simulink model "EV6_LUT_FourWheel_EV6Battery77p4kWh_PowerCorrected"  (R2024a)
settings: Solver=ode4  StartTime=0  StopTime=60  FixedStep=0.001  RelTol=1e-3
PreLoadFcn:
  | VSS_BICYCLE=Simulink.Variant('Dual=0');
  | VSS_DUAL=Simulink.Variant('Dual=1');
  | Dual=1;
  | load('DriveCycle2.mat')
PostLoadFcn:
  | if any(exist('dsrtsu_mdlpostloadfcn', 'file') ~= 0), dsrtsu_mdlpostloadfcn('Execute', bdroot); end
InitFcn:
  | , if any(exist('rtifpga_mdlclblib', 'file') ~= 0), rtifpga_mdlclblib('Init', bdroot); end,
  | , if any(exist('dsmpb_private', 'file') ~= 0), dsmpb_private('dsmpb_mdlclblib', 'Init', bdroot); end,
  | load('DriveCycle2.mat')
model workspace (MAT data in the model file):
  DiffRatio = 10.65
  EV6_2023_BattBranchCapacity_Ah = 55.5236728838
  EV6_2023_BattEnergy_kWh = 77.4
  EV6_2023_BattNominalVoltage_V = 697
  EV6_2023_BattNumCellsParallel = 2
  EV6_2023_BattNumCellsSeries = 192
  EV6_2023_BattOpenVoltCapBpts = [0 0.1 0.2 0.3 0.4 0.5 0.6 0.7 0.8 0.9 1]
  EV6_2023_BattOpenVoltTbl = [2.96762142548 3.40364281191 3.47417488548 3.54470541822 3.61523441014 3.68576186124 3.75628777151 3.82681214095 3.94527005036 4.07101207308 4.2120755254]
  EV6_2023_BattPackCapacity_Ah = 111.047345768
  EV6_2023_BattResistSocBpts = [0 0.2 0.4 0.6 0.8 1]
  EV6_2023_BattResistTbl = [0.0163620057716 0.0118174152018 0.00807187352333 0.00375663957972 0.00266904525531 0.00103635901355 0.0019014404175 0.0172368903217 0.0121226074867 0.00758541551769 0.00474065349228 0.00337561163613 ... (42 elements, 7x6)]
  EV6_2023_BattResistTempBpts = [243.1 253.1 263.1 273.1 283.1 298.1 313.1]
  EV6_2023_InitialPackOCV_V = 726.471714233
  EV6_2023_InitialSOC = 0.638878863672
  EV6_BattCellCapacity_Ah = 60.3
  EV6_BattInitialSOC = 0.638878863672
  EV6_BattOCV_Cell_V = [2.96762142548 3.40364281191 3.47417488548 3.54470541822 3.61523441014 3.68576186124 3.75628777151 3.82681214095 3.94527005036 4.07101207308 4.2120755254]
  EV6_BattOCV_SOC = [0 0.1 0.2 0.3 0.4 0.5 0.6 0.7 0.8 0.9 1]
  EV6_BattPackCapacity_Ah = 120.6
  EV6_BattParallelCells = 2
  EV6_BattResistanceSOC = [0 0.2 0.4 0.6 0.8 1]
  EV6_BattResistanceTable_Ohm = [0.0163620057716 0.0118174152018 0.00807187352333 0.00375663957972 0.00266904525531 0.00103635901355 0.0019014404175 0.0172368903217 0.0121226074867 0.00758541551769 0.00474065349228 0.00337561163613 ... (42 elements, 7x6)]
  EV6_BattResistanceTemp_K = [243.1 253.1 263.1 273.1 283.1 298.1 313.1]
  EV6_BattSeriesCells = 192
  EV6_FinalDriveRatio = 10.65
  EV6_TargetPackResistance_Ohm = 0.132763804608
  Gas = 0.383333333333
undefined symbols (not defined in the file): accel_bp_mps2, AccelCmd, ActTqLF_Nm_, ActTqLR_Nm_, ActTqRF_Nm_, ActTqRR_Nm_, BattChargeLimitMaxPwr, BattChargeLimitSocBpts, BattChargeLimitTbl, BattDischargeLimitSocBpts, BattDischargeLimitTbl, BattDischargeMaxPwr, BrakeMaxPrs, BrakeMaxTrq, ChassisDistCg2FrontAxle, ChassisDistCg2RearAxle, ChassisVehMass, CltchCmd, CoastDown, DecelCmd, DiscIntNeverNeededParam, EnvGravCnst, EnvPrs, EnvTemp, EV6_RegenTorqueGain, EV6_TractionTorqueGain, front_share_regen_3d, front_share_traction_3d, FuelSpecificGrav, GearCmd, h, InitStates, lgSw, limitedMCT, MCT, MtrEffSpdBpts, MtrEffTbl, MtrEffTrqBpts, MtrPwrMax, MtrTrqMax, out_1, pMCT, RealSimPara, Ref_speed, Ref_time, regen_torque_bp_Nm, speed_bp_kph, SteeringCmd, SupvsryCtrlRegenBrkCutOffTbl, SupvsryCtrlRegenSpdBpts, TestScnrioCycleNum, traction_torque_bp_Nm, US06, VEH
libraries: VSIGenLib x65, simulink x54, etargetslib x38, dsmpblib x24, vehdynlibtire x12, autolibshared x11, vehdynlibsuspension x7, vehdynlibtirecommon x7, autolibpowerinfoutils x6, autolibutils x5, autolibsharedcoupling x4, autolibmappedmotor x4
(part 12 of 19)

== system EV6_LUT_FourWheel_EV6Battery77p4kWh_PowerCorrected/Vehicle Under Test1/Vehicle/Driver and Drive Cycle/Driver and PI with FF Control/Speed controller set/In-house CAVE/In-house Speed Controller ==
  note: ToDo: Maybe do something clever with FF and Brake, or maybe not.
      | Bleed FF based on refspd derivative
  RefSpd : Inport
  VehicleSpeed : Inport  Port=2
  Add : Sum  Inputs=+-
  Compare To Constant1 : simulink/Logic and Bit Operations/Compare To Constant  relop=<=  const=0.1  OutDataTypeStr=boolean  ZeroCross=off
  Compare To Constant3 : simulink/Logic and Bit Operations/Compare To Constant  relop=<=  const=0  OutDataTypeStr=boolean  ZeroCross=off
  Constant : Constant  Value=0
  Constant1 : Constant  Value=0
  Detect Fall Negative : simulink/Logic and Bit Operations/Detect Fall Negative  vinit=0  OutDataTypeStr=boolean
  Detect Rise Positive : simulink/Logic and Bit Operations/Detect Rise Positive  vinit=0  OutDataTypeStr=boolean
  Feedforward : Lookup_n-D  Commented=on  NumberOfTableDimensions=1  BreakpointsForDimension1="[0 10    20    30    40    50    60    70    80    90   100   110   120   130   140   150   160]"  Table="[0\t3.5\t12.5\t16\t20\t21\t22\t24.5\t26\t29.5\t32\t33\t34\t36\t37\t38\t39]"  ExtrapMethod=Clip  InternalRulePriority=Speed  RndMeth=Simplest
  Feedforward1 : Lookup_n-D  NumberOfTableDimensions=1  BreakpointsForDimension1="[0 10    20    30    40    50    60    70    80    90   100   110   120   130   140   150   160]"  Table="[0 2.6021    4.7790    6.8575    8.1555    9.4176   10.7914   12.3245   14.1570   15.9699   17.4605   19.0355   21.3079   22.8407   25.3373   26.9453   28.6975]"  ExtrapMethod=Clip  InternalRulePriority=Speed  RndMeth=Simplest
  FeedforwardGain : Gain
  Gain : Gain  Gain=-1
  Ground1 : Ground
  Integrator1 : Integrator  Commented=on
  Ki : Gain
  Kp : Gain  Gain=10
  Limits [-50,50] : Integrator  ExternalReset=either  LimitOutput=on  UpperSaturationLimit=50  LowerSaturationLimit=-50
  Logical Operator : Logic  Operator=OR  Inputs=3  AllPortsSameDT=off  OutDataTypeStr=boolean
  Lowpass Filter : TransferFcn  Denominator=[.02 1]
  Memory : Memory
  Memory1 : Memory
  Min threshold for Brake switch : Constant  Value=0
  Product1 : Product  RndMeth=Zero
  Proportional Gain Scheduling : Lookup_n-D  NumberOfTableDimensions=1  BreakpointsForDimension1=[ 0 30 70]  IndexSearchMethod=Linear search  BeginIndexSearchUsingPreviousIndexResult=on  Table=[1 1 1]  ExtrapMethod=Clip  UseLastTableValue=on  RndMeth=Simplest
  Relational Operator : RelationalOperator  Operator=>  OutDataTypeStr=boolean  InputSameDT=off
  Scope : Scope  NumInputPorts=2
  Scope1 : Scope
  Scope2 : Scope  NumInputPorts=3
  Scope3 : Scope
  Scope4 : Scope  NumInputPorts=2
  Sum : Sum  Inputs=|+-
  Sum1 : Sum  Inputs=+++
  Switch{1..4} (4 alike) : Switch  Criteria=u2 > Threshold  SaturateOnIntegerOverflow=off  InputSameDT=off
  standstill brake [0,100] : Constant  Value=50
  AcceleratorPedalPos : Outport  VectorParamsAs1DForOutWhenUnconnected=off
  BrakePedalPos : Outport  Port=2  VectorParamsAs1DForOutWhenUnconnected=off
  BrakeSwitch : Outport  Port=3  VectorParamsAs1DForOutWhenUnconnected=off
  wires:
  FeedforwardGain/1 -> Sum1/3  "Driver_FdfwdTerm_pct"
  Feedforward1/1 -> FeedforwardGain/1
  Product1/1 -> Sum1/2  "Driver_PropTerm_pct"
  Proportional Gain Scheduling/1 -> Product1/2
  standstill brake [0,100]/1 -> Switch4/1
  Constant/1 -> Switch3/1
  Switch1/1 -> Memory1/1, Scope4/2, Scope2/1, Switch3/3  "AcceleratorPedalPos_pct"
  Compare To Constant1/1 -> Switch4/2, Switch3/2
  Memory1/1 -> Add/1
  Memory/1 -> Add/2
  Add/1 -> Detect Rise Positive/1, Detect Fall Negative/1
  Detect Fall Negative/1 -> Logical Operator/3
  Detect Rise Positive/1 -> Logical Operator/2
  Compare To Constant3/1 -> Logical Operator/1
  Logical Operator/1 -> Limits [-50,50]/2
  Gain/1 -> Switch2/2, Switch2/1
  Ground1/1 -> Switch1/3, Switch2/3
  Sum1/1 -> Switch1/2, Switch1/1, Scope4/1, Gain/1  "Driver_TotCmdPreLim_pct"
  Relational Operator/1 -> Scope2/3, BrakeSwitch/1  "BrakeSwitch"
  Lowpass Filter/1 -> Sum/2, Scope/1  "VS_Flt"
  Switch2/1 -> Memory/1, Scope2/2, Switch4/3, Relational Operator/1  "BrakePedalPosPre_pct"
  VehicleSpeed/1 -> Lowpass Filter/1, Scope/2, Proportional Gain Scheduling/1
  Ki/1 -> Limits [-50,50]/1, Scope3/1  "Driver_IntTerm_pct"
  Sum/1 -> Scope1/1, Ki/1, Kp/1  "SpdErr"
  RefSpd/1 -> Sum/1, Compare To Constant3/1, Compare To Constant1/1, Feedforward1/1  "RefSpd"
  Min threshold for Brake switch/1 -> Relational Operator/2
  Kp/1 -> Product1/1
  Switch3/1 -> AcceleratorPedalPos/1  "AcceleratorPedalPos_pct"
  Switch4/1 -> BrakePedalPos/1  "BrakePedalPos_pct"
  Limits [-50,50]/1 -> Sum1/1  "Driver_IntTerm_pct"

== system EV6_LUT_FourWheel_EV6Battery77p4kWh_PowerCorrected/Vehicle Under Test1/Vehicle/Driver and Drive Cycle/Driver and PI with FF Control/Speed controller set/Predictive/Longitudinal Driver1 ==
  note: To switch variants, right-click on this subsystem (from one level above) and chose:
      | Variant, Active choice, <your selection>
  "Vref " : Inport
  "Vfdbk " : Inport  Port=2
  Longitudinal Driver : Subsystem  VariantControl=0
      mask Display: image('LongitudinalDriver.png', 'center')
  Open Loop : Subsystem  VariantControl=1
      mask Display: disp('Open Loop')
  " OpCmds" : Outport  VectorParamsAs1DForOutWhenUnconnected=off

== system EV6_LUT_FourWheel_EV6Battery77p4kWh_PowerCorrected/Vehicle Under Test1/Vehicle/Driver and Drive Cycle/Driver and PI with FF Control/Speed controller set/Speed tracking controller/In-house CAVE ==
  note: BrakeSwitch
  RefSpd [km/hr] : Inport
  In2 : Inport  Port=2
  Vehicle Speed Controller : Subsystem
  AccelPedalCmd : Outport
  BrakePedalCmd : Outport  Port=2
  Out3 : Outport  Port=3
  wires:
  Vehicle Speed Controller/1(AcceleratorPedalPos) -> AccelPedalCmd/1  "AccelPedalCmd"
  In2/1 -> Vehicle Speed Controller/2(VehicleSpeed)
  RefSpd [km/hr]/1 -> Vehicle Speed Controller/1(RefSpd)
  Vehicle Speed Controller/2(BrakePedalPos) -> BrakePedalCmd/1  "BrakePedalCmd"
  Vehicle Speed Controller/3(BrakeSwitch) -> Out3/1

== system EV6_LUT_FourWheel_EV6Battery77p4kWh_PowerCorrected/Vehicle Under Test1/Vehicle/Driver and Drive Cycle/Driver and PI with FF Control/Speed controller set/Speed tracking controller/PIF ==
  RefSpd [km/hr] : Inport
  In2 : Inport  Port=2
  Compare To Constant1 : simulink/Logic and Bit Operations/Compare To Constant  relop=<=  const=0.1  OutDataTypeStr=boolean  ZeroCross=off
  Constant : Constant  Value=0
  Constant1 : Constant  Value=0
  Gain : Gain  Gain=1/3.6
  Gain1 : Gain  Gain=1/3.6
  Gain2 : Gain  Gain=100
  Gain3 : Gain  Gain=100
  Longitudinal Driver : autolibshared/Longitudinal Driver  extAccelOvr=off  extDecelOvr=off  extAccelHld=off  extDecelHld=off  extAccelZero=off  extDecelZero=off  cntrlType=PI  shftType=None  velUnits=m/s  gearOut=off  Kp=2  Ki=2  Kff=.1*0.4  Kg=0  VehVelVec=[0 100]  KffVec=[.1 .1]  KpVec=[10 10]  KiVec=[5 5]  KgVec=[0 0]  m=1500  Kpt=3000  tau=.1  L=2  aR=200  bR=2.5  cR=.5  g=9.81  vnom=1  Kaw=1  tauerr=.01  tauPt=2  GearInit=0  tShift=.1  pdlVec=[0.1 0.4 0.5 0.9]  upShftTbl=[-1 12.9375 26.4375 39.9375 51.18749999999999 62.4375 72.84375 83.25;-1 16.3125 29.8125 43.3125 54.5624 65.8125 76.78125 87.75;-1 19.6875 33.1875 46.68749999999999 57.9375 69.1875 80.71875 92.25;-1 33 52.5 77.25 100.5 138.75 161.875 185]  dwnShftTbl=[1 9.5625 23.0625 36.5625 47.8125 59.0625 68.90625 78.75;1 12.9375 26.4375 39.9375 51.18749999999999 62.4375 72.84375 83.25;1 16.3125 29.8125 43.3125 54.562499 65.8125 76.78125 87.75;1 19.6875 33.1875 46.68749999999999 57.9375 69.1875 80.71875 92.25]  tClutch=.5  tRev=.5  tPark=120  aMode=2  UpGearVec="[0  1  2  3  4  5  6  7]"  DownGearVec="[1  2  3  4  5  6  7  8]"
      settings: LibrarySourceBlock=vehdynlibdriver/Longitudinal Driver
  Lowpass Filter : TransferFcn  Denominator=[.01 1]
  Min threshold for Brake switch : Constant  Value=0
  Relational Operator : RelationalOperator  Operator=>  OutDataTypeStr=boolean  InputSameDT=off
  Switch3 : Switch  Criteria=u2 > Threshold  SaturateOnIntegerOverflow=off  InputSameDT=off
  Switch4 : Switch  Criteria=u2 > Threshold  SaturateOnIntegerOverflow=off  InputSameDT=off
  Terminator : Terminator
  standstill brake [0,1] : Constant  Value=0.5
  AccelPedalCmd : Outport
  BrakePedalCmd : Outport  Port=2
  Out3 : Outport  Port=3
  wires:
  Lowpass Filter/1 -> Gain1/1  "VS_Flt"
  Switch4/1 -> Gain3/1  "BrakePedalPos_pct"
  Switch3/1 -> Gain2/1  "AcceleratorPedalPos_pct"
  standstill brake [0,1]/1 -> Switch4/1
  Compare To Constant1/1 -> Switch3/2, Switch4/2
  Constant/1 -> Switch3/1
  Longitudinal Driver/2 -> Switch3/3  "AcceleratorPedalPosPre_pct"
  Longitudinal Driver/1 -> Terminator/1
  Gain2/1 -> AccelPedalCmd/1  "AccelPedalCmd"
  Gain3/1 -> BrakePedalCmd/1  "BrakePedalCmd"
  In2/1 -> Lowpass Filter/1
  RefSpd [km/hr]/1 -> Gain/1
  Constant1/1 -> Longitudinal Driver/3
  Gain/1 -> Longitudinal Driver/1, Compare To Constant1/1
  Longitudinal Driver/3 -> Relational Operator/1, Switch4/3  "BrakePedalPosPre_pct"
  Relational Operator/1 -> Out3/1  "BrakeSwitch"
  Min threshold for Brake switch/1 -> Relational Operator/2
  Gain1/1 -> Longitudinal Driver/2

== system EV6_LUT_FourWheel_EV6Battery77p4kWh_PowerCorrected/Vehicle Under Test1/Vehicle/Driver and Drive Cycle/Driver and PI with FF Control/Speed controller set/Speed tracking controller/Predictive ==
  RefSpd [km/hr] : Inport
  In2 : Inport  Port=2
  Compare To Constant1 : simulink/Logic and Bit Operations/Compare To Constant  relop=<=  const=0.1  OutDataTypeStr=boolean  ZeroCross=off
  Constant : Constant  Value=0
  Constant1 : Constant  Value=0
  Gain : Gain  Gain=1/3.6
  Gain1 : Gain  Gain=1/3.6
  Gain4 : Gain  Gain=100
  Gain5 : Gain  Gain=100
  Longitudinal Driver : autolibshared/Longitudinal Driver  extAccelOvr=off  extDecelOvr=off  extAccelHld=off  extDecelHld=off  extAccelZero=off  extDecelZero=off  cntrlType=Predictive  shftType=None  velUnits=m/s  gearOut=off  Kp=10  Ki=5  Kff=.1  Kg=0  VehVelVec=[0 100]  KffVec=[.1 .1]  KpVec=[10 10]  KiVec=[5 5]  KgVec=[0 0]  m=2040  Kpt=6200  tau=0.1  L=3  aR=200/10  bR=2.5/10  cR=.3  g=9.807  vnom=5  Kaw=1  tauerr=.01  tauPt=2  GearInit=0  tShift=.1  pdlVec=[0.1 0.4 0.5 0.9]  upShftTbl=[-1 12.9375 26.4375 39.9375 51.18749999999999 62.4375 72.84375 83.25;-1 16.3125 29.8125 43.3125 54.5624 65.8125 76.78125 87.75;-1 19.6875 33.1875 46.68749999999999 57.9375 69.1875 80.71875 92.25;-1 33 52.5 77.25 100.5 138.75 161.875 185]  dwnShftTbl=[1 9.5625 23.0625 36.5625 47.8125 59.0625 68.90625 78.75;1 12.9375 26.4375 39.9375 51.18749999999999 62.4375 72.84375 83.25;1 16.3125 29.8125 43.3125 54.562499 65.8125 76.78125 87.75;1 19.6875 33.1875 46.68749999999999 57.9375 69.1875 80.71875 92.25]  tClutch=.5  tRev=.5  tPark=120  aMode=2  UpGearVec="[0  1  2  3  4  5  6  7]"  DownGearVec="[1  2  3  4  5  6  7  8]"
      settings: LibrarySourceBlock=vehdynlibdriver/Longitudinal Driver
  Lowpass Filter : TransferFcn  Denominator=[.02 1]
  Min threshold for Brake switch : Constant  Value=0
  Relational Operator : RelationalOperator  Operator=>  OutDataTypeStr=boolean  InputSameDT=off
  Switch3 : Switch  Criteria=u2 > Threshold  SaturateOnIntegerOverflow=off  InputSameDT=off
  Switch4 : Switch  Criteria=u2 > Threshold  SaturateOnIntegerOverflow=off  InputSameDT=off
  Terminator : Terminator
  standstill brake [0,1] : Constant  Value=0.5
  AccelPedalCmd : Outport
  BrakePedalCmd : Outport  Port=2
  Out3 : Outport  Port=3
  wires:
  Lowpass Filter/1 -> Gain1/1  "VS_Flt"
  Longitudinal Driver/2 -> Switch3/3  "AcceleratorPedalPosPre_pct"
  Gain5/1 -> BrakePedalCmd/1  "BrakePedalCmd"
  Gain/1 -> Longitudinal Driver/1, Compare To Constant1/1
  Gain4/1 -> AccelPedalCmd/1  "AccelPedalCmd"
  Constant/1 -> Switch3/1
  Compare To Constant1/1 -> Switch3/2, Switch4/2
  Switch3/1 -> Gain4/1  "AcceleratorPedalPos_pct"
  Switch4/1 -> Gain5/1  "BrakePedalPos_pct"
  Longitudinal Driver/3 -> Relational Operator/1, Switch4/3  "BrakePedalPosPre_pct"
  standstill brake [0,1]/1 -> Switch4/1
  Longitudinal Driver/1 -> Terminator/1
  In2/1 -> Lowpass Filter/1
  RefSpd [km/hr]/1 -> Gain/1
  Constant1/1 -> Longitudinal Driver/3
  Relational Operator/1 -> Out3/1  "BrakeSwitch"
  Min threshold for Brake switch/1 -> Relational Operator/2
  Gain1/1 -> Longitudinal Driver/2

== system EV6_LUT_FourWheel_EV6Battery77p4kWh_PowerCorrected/Vehicle Under Test1/Vehicle/Powertrain Supervisory Controller /Engine Torque Command/Motor Torque Arbitration and Power Management/Power Management/Check Within Limits ==
  up : Inport
  u : Inport  Port=2
  lo : Inport  Port=3
  Compare To Zero : simulink/Logic and Bit Operations/Compare To Zero  relop=>=  OutDataTypeStr=boolean
  Compare To Zero1 : simulink/Logic and Bit Operations/Compare To Zero  relop=<=  OutDataTypeStr=boolean
  Logical Operator : Logic  AllPortsSameDT=off  OutDataTypeStr=boolean
  Saturation Dynamic1 : simulink/Discontinuities/Saturation Dynamic  OutMin=[]  OutMax=[]  OutDataTypeStr=Inherit: Same as second input  OutDataType=fixdt(1, 16)  OutScaling=2^-10  DoSatur=off
  Subtract : Sum  Inputs=+-
  Subtract1 : Sum  Inputs=-+
  InLimit : Outport  VectorParamsAs1DForOutWhenUnconnected=off
  y : Outport  Port=2  VectorParamsAs1DForOutWhenUnconnected=off
  wires:
  Saturation Dynamic1/1 -> y/1
  lo/1 -> Subtract1/2, Saturation Dynamic1/3
  up/1 -> Subtract/1, Saturation Dynamic1/1
  u/1 -> Subtract1/1, Subtract/2, Saturation Dynamic1/2
  Subtract/1 -> Compare To Zero/1
  Subtract1/1 -> Compare To Zero1/1
  Compare To Zero/1 -> Logical Operator/1
  Compare To Zero1/1 -> Logical Operator/2
  Logical Operator/1 -> InLimit/1

== system EV6_LUT_FourWheel_EV6Battery77p4kWh_PowerCorrected/Vehicle Under Test1/Vehicle/Powertrain Supervisory Controller /Engine Torque Command/Motor Torque Arbitration and Power Management/Power Management/Mech to Elec Power Estimate ==
  note: Check if Motoring
      | or Generating
  note: Using an Efficiency Map, we can estimate the
      | Electric Power from the Mechanical  Torque Request.
  note: Pelec_req = Pmech_req*Eff^k,
      | k = -1 if Motoring >= 0,
      | k = 1 if Generating < 0
  MotTrqCmd : Inport
  MotSpd : Inport  Port=2
  Abs : Abs  SaturateOnIntegerOverflow=off
  Abs1 : Abs  SaturateOnIntegerOverflow=off
  Constant1 : Constant  Value=-1  SampleTime=-1
  Constant2 : Constant  SampleTime=-1
  Eff Map : Lookup_n-D  BreakpointsForDimension1=MtrEffSpdBpts  BreakpointsForDimension2=MtrEffTrqBpts  Table=MtrEffTbl  ExtrapMethod=Clip  UseLastTableValue=on  InternalRulePriority=Speed  OutDataTypeStr=Inherit: Inherit from 'Table data'  RndMeth=Simplest
      settings: InputPortMap=u0,u1
  Gain1 : Gain  Gain=1/100
  Math Function : Math  Operator=pow  SignedPower=on  OutputSignalType=real
  Product : Product
  Product3 : Product
  Product4 : Product
  Switch2 : Switch  SaturateOnIntegerOverflow=off  InputSameDT=off
  rads_to_rpm : Gain  Gain=30/pi
  MotPwrElecReq : Outport  VectorParamsAs1DForOutWhenUnconnected=off
  Eff2k : Outport  Port=2  VectorParamsAs1DForOutWhenUnconnected=off
  wires:
  Product3/1 -> Product4/1
  Switch2/1 -> Math Function/2
  Constant1/1 -> Switch2/1
  Constant2/1 -> Switch2/3
  Eff Map/1 -> Gain1/1
  Abs/1 -> Eff Map/1
  Gain1/1 -> Math Function/1
  Math Function/1 -> Eff2k/1, Product4/2
  Product4/1 -> MotPwrElecReq/1
  Abs1/1 -> Eff Map/2
  rads_to_rpm/1 -> Abs/1
  Product/1 -> Switch2/2
  MotSpd/1 -> Product3/1, Product/1, rads_to_rpm/1
  MotTrqCmd/1 -> Product3/2, Product/2, Abs1/1

== system EV6_LUT_FourWheel_EV6Battery77p4kWh_PowerCorrected/Vehicle Under Test1/Vehicle/Powertrain Supervisory Controller /Engine Torque Command/Motor Torque Arbitration and Power Management/Power Management/Torque Limit ==
  MotTrq : Inport
  MotSpd : Inport  Port=2
  Gain : Gain  Gain=-1
  Max Motor Torque : LibPtSupervisoryCtrl/Powertrain Supervisory Controller /Engine Torque Command/Accel Pedal to Traction Wheel Torque Request/Max Motor Torque  SystemSampleTime=-1  VariantActivationTime=update diagram  AllowFlexibleInterface=on  Latency=0  AutoFrameSizeCalculation=off
  Saturation Dynamic : simulink/Discontinuities/Saturation Dynamic  OutMin=[]  OutMax=[]  OutDataTypeStr=Inherit: Same as second input  OutDataType=fixdt(1, 16)  OutScaling=2^-10  DoSatur=off
  MotTrqCmd : Outport  VectorParamsAs1DForOutWhenUnconnected=off
  wires:
  MotTrq/1 -> Saturation Dynamic/2
  Saturation Dynamic/1 -> MotTrqCmd/1
  Max Motor Torque/1 -> Gain/1, Saturation Dynamic/1
  Gain/1 -> Saturation Dynamic/3
  MotSpd/1 -> Max Motor Torque/1

== system EV6_LUT_FourWheel_EV6Battery77p4kWh_PowerCorrected/Vehicle Under Test1/Vehicle/Rototest and ORNL Interface/Get Wheel Spd Cmd Based on Wheel Dynamics/Whl Dynamics & Format CM Powertrain Signal/Subsystem/WheelInertia ==
  In1 : Inport
  Divide : Product  Inputs=*/
  Switch : Switch  Criteria=u2 ~= 0  ZeroCross=off  SaturateOnIntegerOverflow=off  InputSameDT=off
  Zero : Constant
  Zero1 : Constant  Value=0.74063
  Out1 : Outport
  wires:
  Divide/1 -> Out1/1
  In1/1 -> Divide/1
  Zero/1 -> Switch/3
  Switch/1 -> Divide/2
  Zero1/1 -> Switch/2, Switch/1

== system EV6_LUT_FourWheel_EV6Battery77p4kWh_PowerCorrected/Vehicle Under Test1/Vehicle/Rototest and ORNL Interface/Get Wheel Spd Cmd Based on Wheel Dynamics/Whl Dynamics & Format CM Powertrain Signal/Subsystem/WheelInertia1 ==
  In1 : Inport
  Divide : Product  Inputs=*/
  Switch : Switch  Criteria=u2 ~= 0  ZeroCross=off  SaturateOnIntegerOverflow=off  InputSameDT=off
  Zero : Constant
  Zero1 : Constant  Value=0.82
  axleTorq : Outport
  wires:
  Divide/1 -> axleTorq/1
  In1/1 -> Divide/1
  Zero/1 -> Switch/3
  Switch/1 -> Divide/2
  Zero1/1 -> Switch/2, Switch/1

== system EV6_LUT_FourWheel_EV6Battery77p4kWh_PowerCorrected/Vehicle Under Test1/Vehicle/Rototest and ORNL Interface/Get Wheel Spd Cmd Based on Wheel Dynamics/Whl Dynamics & Format CM Powertrain Signal/Subsystem1/WheelInertia ==
  In1 : Inport
  Divide : Product  Inputs=*/
  Read CM Parameter : CarMaker4SL/Read CM Parameter  xfile=Vehicle  xkey=Wheel.fl.I  xnout=3  xdefaults=[]  xmuxed=off  xstime=Continuous
      settings: SourceProductName=CarMaker4SL
  Switch : Switch  Criteria=u2 ~= 0  ZeroCross=off  SaturateOnIntegerOverflow=off  InputSameDT=off
  Terminator : Terminator
  Terminator1 : Terminator
  Zero : Constant
  Out1 : Outport
  wires:
  Divide/1 -> Out1/1
  Read CM Parameter/1 -> Terminator/1
  Read CM Parameter/3 -> Terminator1/1
  In1/1 -> Divide/1
  Zero/1 -> Switch/3
  Switch/1 -> Divide/2
  Read CM Parameter/2 -> Switch/2, Switch/1

== system EV6_LUT_FourWheel_EV6Battery77p4kWh_PowerCorrected/Vehicle Under Test1/Vehicle/Rototest and ORNL Interface/Get Wheel Spd Cmd Based on Wheel Dynamics/Whl Dynamics & Format CM Powertrain Signal/Subsystem2/WheelInertia ==
  In1 : Inport
  Divide : Product  Inputs=*/
  Switch : Switch  Criteria=u2 ~= 0  ZeroCross=off  SaturateOnIntegerOverflow=off  InputSameDT=off
  Zero : Constant
  Zero1 : Constant  Value=0.74063
  Out1 : Outport
  wires:
  Divide/1 -> Out1/1
  In1/1 -> Divide/1
  Zero/1 -> Switch/3
  Switch/1 -> Divide/2
  Zero1/1 -> Switch/2, Switch/1

== system EV6_LUT_FourWheel_EV6Battery77p4kWh_PowerCorrected/Vehicle Under Test1/Vehicle/Rototest and ORNL Interface/Get Wheel Spd Cmd Based on Wheel Dynamics/Whl Dynamics & Format CM Powertrain Signal/Subsystem2/WheelInertia1 ==
  In1 : Inport
  Divide : Product  Inputs=*/
  Switch : Switch  Criteria=u2 ~= 0  ZeroCross=off  SaturateOnIntegerOverflow=off  InputSameDT=off
  Zero : Constant
  Zero1 : Constant  Value=0.82
  Out1 : Outport
  wires:
  Divide/1 -> Out1/1
  In1/1 -> Divide/1
  Zero/1 -> Switch/3
  Switch/1 -> Divide/2
  Zero1/1 -> Switch/2, Switch/1

== system EV6_LUT_FourWheel_EV6Battery77p4kWh_PowerCorrected/Vehicle Under Test1/Vehicle/Rototest and ORNL Interface/Get Wheel Spd Cmd Based on Wheel Dynamics/Whl Dynamics & Format CM Powertrain Signal/Subsystem3/WheelInertia ==
  In1 : Inport
  Divide : Product  Inputs=*/
  Switch : Switch  Criteria=u2 ~= 0  ZeroCross=off  SaturateOnIntegerOverflow=off  InputSameDT=off
  Zero : Constant
  Zero1 : Constant  Value=0.74063
  Out1 : Outport
  wires:
  Divide/1 -> Out1/1
  In1/1 -> Divide/1
  Zero/1 -> Switch/3
  Switch/1 -> Divide/2
  Zero1/1 -> Switch/2, Switch/1

== system EV6_LUT_FourWheel_EV6Battery77p4kWh_PowerCorrected/Vehicle Under Test1/Vehicle/Rototest and ORNL Interface/Get Wheel Spd Cmd Based on Wheel Dynamics/Whl Dynamics & Format CM Powertrain Signal/Subsystem3/WheelInertia1 ==
  In1 : Inport
  Divide : Product  Inputs=*/
  Switch : Switch  Criteria=u2 ~= 0  ZeroCross=off  SaturateOnIntegerOverflow=off  InputSameDT=off
  Zero : Constant
  Zero1 : Constant  Value=0.82
  axleTorq : Outport
  wires:
  Divide/1 -> axleTorq/1
  In1/1 -> Divide/1
  Zero/1 -> Switch/3
  Switch/1 -> Divide/2
  Zero1/1 -> Switch/2, Switch/1

== system EV6_LUT_FourWheel_EV6Battery77p4kWh_PowerCorrected/Vehicle Under Test1/Vehicle/Rototest and ORNL Interface/Get Wheel Spd Cmd Based on Wheel Dynamics/Whl Dynamics & Format CM Powertrain Signal/Subsystem4/WheelInertia ==
  In1 : Inport
  Divide : Product  Inputs=*/
  Switch : Switch  Criteria=u2 ~= 0  ZeroCross=off  SaturateOnIntegerOverflow=off  InputSameDT=off
  Zero : Constant
  Zero1 : Constant  Value=0.74063
  Out1 : Outport
  wires:
  Divide/1 -> Out1/1
  In1/1 -> Divide/1
  Zero/1 -> Switch/3
  Switch/1 -> Divide/2
  Zero1/1 -> Switch/2, Switch/1

== system EV6_LUT_FourWheel_EV6Battery77p4kWh_PowerCorrected/Vehicle Under Test1/Vehicle/Rototest and ORNL Interface/Get Wheel Spd Cmd Based on Wheel Dynamics/Whl Dynamics & Format CM Powertrain Signal/Subsystem4/WheelInertia1 ==
  In1 : Inport
  Divide : Product  Inputs=*/
  Switch : Switch  Criteria=u2 ~= 0  ZeroCross=off  SaturateOnIntegerOverflow=off  InputSameDT=off
  Zero : Constant
  Zero1 : Constant  Value=0.82
  axleTorq : Outport
  wires:
  Divide/1 -> axleTorq/1
  In1/1 -> Divide/1
  Zero/1 -> Switch/3
  Switch/1 -> Divide/2
  Zero1/1 -> Switch/2, Switch/1

== system EV6_LUT_FourWheel_EV6Battery77p4kWh_PowerCorrected/Vehicle Under Test1/Vehicle/Rototest and ORNL Interface/Get Wheel Spd Cmd Based on Wheel Dynamics/Whl Dynamics & Format CM Powertrain Signal/Subsystem5/WheelInertia1 ==
  In1 : Inport
  Divide : Product  Inputs=*/
  Read CM Parameter : CarMaker4SL/Read CM Parameter  xfile=Vehicle  xkey=Wheel.fr.I  xnout=3  xdefaults=[]  xmuxed=off  xstime=Continuous
      settings: SourceProductName=CarMaker4SL
  Switch : Switch  Criteria=u2 ~= 0  ZeroCross=off  SaturateOnIntegerOverflow=off  InputSameDT=off
  Terminator : Terminator
  Terminator1 : Terminator
  Zero : Constant
  Out1 : Outport
  wires:
  Switch/1 -> Divide/2
  Zero/1 -> Switch/3
  Read CM Parameter/2 -> Switch/1, Switch/2
  In1/1 -> Divide/1
  Read CM Parameter/3 -> Terminator1/1
  Read CM Parameter/1 -> Terminator/1
  Divide/1 -> Out1/1

== system EV6_LUT_FourWheel_EV6Battery77p4kWh_PowerCorrected/Vehicle Under Test1/Vehicle/Rototest and ORNL Interface/Get Wheel Spd Cmd Based on Wheel Dynamics/Whl Dynamics & Format CM Powertrain Signal/Subsystem6/WheelInertia2 ==
  In1 : Inport
  Divide : Product  Inputs=*/
  Read CM Parameter : CarMaker4SL/Read CM Parameter  xfile=Vehicle  xkey=Wheel.rl.I  xnout=3  xdefaults=[]  xmuxed=off  xstime=Continuous
      settings: SourceProductName=CarMaker4SL
  Switch : Switch  Criteria=u2 ~= 0  ZeroCross=off  SaturateOnIntegerOverflow=off  InputSameDT=off
  Terminator : Terminator
  Terminator1 : Terminator
  Zero : Constant
  Out1 : Outport
  wires:
  Divide/1 -> Out1/1
  Read CM Parameter/1 -> Terminator/1
  Read CM Parameter/3 -> Terminator1/1
  In1/1 -> Divide/1
  Read CM Parameter/2 -> Switch/2, Switch/1
  Zero/1 -> Switch/3
  Switch/1 -> Divide/2

== system EV6_LUT_FourWheel_EV6Battery77p4kWh_PowerCorrected/Vehicle Under Test1/Vehicle/Rototest and ORNL Interface/Get Wheel Spd Cmd Based on Wheel Dynamics/Whl Dynamics & Format CM Powertrain Signal/Subsystem7/WheelInertia3 ==
  In1 : Inport
  Divide : Product  Inputs=*/
  Read CM Parameter : CarMaker4SL/Read CM Parameter  xfile=Vehicle  xkey=Wheel.rr.I  xnout=3  xdefaults=[]  xmuxed=off  xstime=Continuous
      settings: SourceProductName=CarMaker4SL
  Switch : Switch  Criteria=u2 ~= 0  ZeroCross=off  SaturateOnIntegerOverflow=off  InputSameDT=off
  Terminator : Terminator
  Terminator1 : Terminator
  Zero : Constant
  Out1 : Outport
  wires:
  Switch/1 -> Divide/2
  Zero/1 -> Switch/3
  Read CM Parameter/2 -> Switch/1, Switch/2
  In1/1 -> Divide/1
  Read CM Parameter/3 -> Terminator1/1
  Read CM Parameter/1 -> Terminator/1
  Divide/1 -> Out1/1

== system EV6_LUT_FourWheel_EV6Battery77p4kWh_PowerCorrected/Vehicle Under Test1/Vehicle/Rototest and ORNL Interface/To Rototest with Band-Aid/Logging/RotoTestEthRXLogging/Depacker ==
  SysStsBits : Inport
  Extract Bits1 : simulink/Logic and Bit Operations/Extract Bits  bitsToExtract=Range of bits  numBits=8  bitIdxRange=[7]  outScalingMode=Preserve fixed-point scaling
  Extract Bits10 : simulink/Logic and Bit Operations/Extract Bits  bitsToExtract=Range of bits  numBits=8  bitIdxRange=[9]  outScalingMode=Preserve fixed-point scaling
  Extract Bits11 : simulink/Logic and Bit Operations/Extract Bits  bitsToExtract=Range of bits  numBits=8  bitIdxRange=[10]  outScalingMode=Preserve fixed-point scaling
  Extract Bits12 : simulink/Logic and Bit Operations/Extract Bits  bitsToExtract=Range of bits  numBits=8  bitIdxRange=[11]  outScalingMode=Preserve fixed-point scaling
  Extract Bits13 : simulink/Logic and Bit Operations/Extract Bits  bitsToExtract=Range of bits  numBits=8  bitIdxRange=[12]  outScalingMode=Preserve fixed-point scaling
  Extract Bits14 : simulink/Logic and Bit Operations/Extract Bits  bitsToExtract=Range of bits  numBits=8  bitIdxRange=[13]  outScalingMode=Preserve fixed-point scaling
  Extract Bits15 : simulink/Logic and Bit Operations/Extract Bits  bitsToExtract=Range of bits  numBits=8  bitIdxRange=[14]  outScalingMode=Preserve fixed-point scaling
  Extract Bits16 : simulink/Logic and Bit Operations/Extract Bits  bitsToExtract=Range of bits  numBits=8  bitIdxRange=[15]  outScalingMode=Preserve fixed-point scaling
  Extract Bits2 : simulink/Logic and Bit Operations/Extract Bits  bitsToExtract=Range of bits  numBits=8  bitIdxRange=[6]  outScalingMode=Preserve fixed-point scaling
  Extract Bits3 : simulink/Logic and Bit Operations/Extract Bits  bitsToExtract=Range of bits  numBits=8  bitIdxRange=[5]  outScalingMode=Preserve fixed-point scaling
  Extract Bits4 : simulink/Logic and Bit Operations/Extract Bits  bitsToExtract=Range of bits  numBits=8  bitIdxRange=[4]  outScalingMode=Preserve fixed-point scaling
  Extract Bits5 : simulink/Logic and Bit Operations/Extract Bits  bitsToExtract=Range of bits  numBits=8  bitIdxRange=[3]  outScalingMode=Preserve fixed-point scaling
  Extract Bits6 : simulink/Logic and Bit Operations/Extract Bits  bitsToExtract=Range of bits  numBits=8  bitIdxRange=[2]  outScalingMode=Preserve fixed-point scaling
  Extract Bits7 : simulink/Logic and Bit Operations/Extract Bits  bitsToExtract=Range of bits  numBits=8  bitIdxRange=[1]  outScalingMode=Preserve fixed-point scaling
  Extract Bits8 : simulink/Logic and Bit Operations/Extract Bits  bitsToExtract=Range of bits  numBits=8  bitIdxRange=[0]  outScalingMode=Preserve fixed-point scaling
  Extract Bits9 : simulink/Logic and Bit Operations/Extract Bits  bitsToExtract=Range of bits  numBits=8  bitIdxRange=[8]  outScalingMode=Preserve fixed-point scaling
  Gain : Gain  Gain=1/128
  Gain1 : Gain  Gain=1/64
  Gain10 : Gain  Gain=1/1024
  Gain11 : Gain  Gain=1/2048
  Gain12 : Gain  Gain=1/4096
  Gain13 : Gain  Gain=1/8192
  Gain14 : Gain  Gain=1/16384
  Gain15 : Gain  Gain=1/32768
  Gain2 : Gain  Gain=1/32
  Gain3 : Gain  Gain=1/16
  Gain4 : Gain  Gain=1/8
  Gain5 : Gain  Gain=1/4
  Gain6 : Gain  Gain=1/2
  Gain7 : Gain  Gain=1/1
  Gain8 : Gain  Gain=1/256
  Gain9 : Gain  Gain=1/512
  Header : VSIGenLib/Header  not=''
  Terminator{,1..11} (12 alike) : Terminator
  FaultActive : Outport
  WarningsActive : Outport  Port=2
  MeasuringStatus : Outport  Port=3
  SystemActive : Outport  Port=4
  wires:
  Extract Bits10/1 -> Gain9/1
  Extract Bits11/1 -> Gain10/1
  Extract Bits12/1 -> Gain11/1
  Gain10/1 -> Terminator3/1  "Reserved"
  Gain9/1 -> Terminator4/1  "Reserved"
  Gain12/1 -> Terminator1/1  "Reserved"
  Gain11/1 -> Terminator2/1  "Reserved"
  Gain13/1 -> Terminator/1  "Reserved"
  Gain14/1 -> WarningsActive/1  "WarningsActive"
  Gain15/1 -> FaultActive/1  "FaultActive"
  Extract Bits13/1 -> Gain12/1
  Extract Bits14/1 -> Gain13/1
  Extract Bits15/1 -> Gain14/1
  Extract Bits16/1 -> Gain15/1
  Gain8/1 -> Terminator5/1  "Reserved"
  Extract Bits9/1 -> Gain8/1
  Gain7/1 -> SystemActive/1  "SystemActive"
  Gain6/1 -> MeasuringStatus/1  "MeasuringStatus"
  Gain5/1 -> Terminator11/1  "Reserved"
  Gain4/1 -> Terminator10/1  "Reserved"
  Gain3/1 -> Terminator9/1  "Reserved"
  Gain1/1 -> Terminator7/1  "Reserved"
  Gain2/1 -> Terminator8/1  "Reserved"
  Gain/1 -> Terminator6/1  "Reserved"
  Extract Bits5/1 -> Gain4/1
  Extract Bits7/1 -> Gain6/1
  SysStsBits/1 -> Extract Bits9/1, Extract Bits10/1, Extract Bits16/1, Extract Bits15/1, Extract Bits14/1, Extract Bits13/1, Extract Bits12/1, Extract Bits11/1, Extract Bits8/1, Extract Bits7/1, Extract Bits6/1, Extract Bits5/1, Extract Bits4/1, Extract Bits3/1, Extract Bits2/1, Extract Bits1/1
  Extract Bits4/1 -> Gain3/1
  Extract Bits1/1 -> Gain/1
  Extract Bits8/1 -> Gain7/1
  Extract Bits3/1 -> Gain2/1
  Extract Bits6/1 -> Gain5/1
  Extract Bits2/1 -> Gain1/1

== system EV6_LUT_FourWheel_EV6Battery77p4kWh_PowerCorrected/Vehicle Under Test1/Vehicle/Vehicle Dynamics/Vehicle 14DOF/Suspension/Double Wishbone Suspension/Steer Rate Adapter ==
  Veh : Inport
  Add : Sum
  Bus Selector3 : BusSelector  OutputSignals=BdyFrm.Cg.AngVel.r
  Constant : Constant  Value=zeros(1,4)
  Matrix Concatenate : Concatenate  NumInputs=3  Mode=Multidimensional array
  Matrix Concatenate1 : Concatenate  NumInputs=3  Mode=Multidimensional array
  Reshape2 : Reshape  OutputDimensionality=Row vector (2-D)
  Reshape3 : Reshape  OutputDimensionality=Row vector (2-D)
  Reshape4 : Reshape  OutputDimensionality=Row vector (2-D)
  Selector3 : Selector  InputPortWidth=1  IndexOptions=Index vector (dialog)  Indices=[1 1 1 1]  OutputSizes=1
  SteerRates : Constant  Value=zeros(1,4)
  AngVel : Outport  VectorParamsAs1DForOutWhenUnconnected=off
  wires:
  Add/1 -> AngVel/1  "AngVel"
  Veh/1 -> Bus Selector3/1
  Matrix Concatenate1/1 -> Add/1
  Reshape3/1 -> Matrix Concatenate/1, Matrix Concatenate/2
  Reshape4/1 -> Matrix Concatenate/3
  SteerRates/1 -> Reshape2/1
  Matrix Concatenate/1 -> Add/2
  Bus Selector3/1 -> Selector3/1  "<r>"
  Selector3/1 -> Reshape4/1
  Constant/1 -> Reshape3/1
  Reshape2/1 -> Matrix Concatenate1/2, Matrix Concatenate1/3, Matrix Concatenate1/1

== system EV6_LUT_FourWheel_EV6Battery77p4kWh_PowerCorrected/Vehicle Under Test1/Vehicle/Vehicle Dynamics/Vehicle 14DOF/Suspension/Double Wishbone Suspension/Steering Adapter ==
  Steer : Inport
  Reshape1 : Reshape  OutputDimensionality=Row vector (2-D)
  Selector : Selector  IndexOptions=Index vector (dialog)  Indices=[1 2]  OutputSizes=1
  StrgAng : Outport  VectorParamsAs1DForOutWhenUnconnected=off
  wires:
  Selector/1 -> Reshape1/1
  Steer/1 -> Selector/1
  Reshape1/1 -> StrgAng/1

== system EV6_LUT_FourWheel_EV6Battery77p4kWh_PowerCorrected/Vehicle Under Test1/Vehicle/Vehicle Dynamics/Vehicle 14DOF/Suspension/Double Wishbone Suspension/Vehicle Adapter ==
  Veh : Inport
  Bus Creator3 : BusCreator  Inputs=2
  Bus Selector1 : BusSelector  OutputSignals=InertFrm.FrntAxl.Lft.Disp.X,InertFrm.FrntAxl.Lft.Disp.Y,InertFrm.FrntAxl.Lft.Disp.Z,InertFrm.FrntAxl.Rght.Disp.X,InertFrm.FrntAxl.Rght.Disp.Y,InertFrm.FrntAxl.Rght.Disp.Z,InertFrm.RearAxl.Lft.Disp.X,InertFrm.RearAxl.Lft.Disp.Y,InertFrm.RearAxl.Lft.Disp.Z,InertFrm.RearAxl.Rght.Disp.X,InertFrm.RearAxl.Rght.Disp.Y,InertFrm.RearAxl.Rght.Disp.Z
  Bus Selector2 : BusSelector  OutputSignals=BdyFrm.FrntAxl.Lft.Vel.xdot,BdyFrm.FrntAxl.Lft.Vel.ydot,BdyFrm.FrntAxl.Lft.Vel.zdot,BdyFrm.FrntAxl.Rght.Vel.xdot,BdyFrm.FrntAxl.Rght.Vel.ydot,BdyFrm.FrntAxl.Rght.Vel.zdot,BdyFrm.RearAxl.Lft.Vel.xdot,BdyFrm.RearAxl.Lft.Vel.ydot,BdyFrm.RearAxl.Lft.Vel.zdot,BdyFrm.RearAxl.Rght.Vel.xdot,BdyFrm.RearAxl.Rght.Vel.ydot,BdyFrm.RearAxl.Rght.Vel.zdot
  Inertial Frame CG to Axle Offset : Constant  Value=[zeros(2,4);h*ones(1,4)+VEH.InitialVertPosition*0]
  Mux1 : Mux  Inputs=12
  Mux2 : Mux  Inputs=12
  Reshape1 : Reshape  OutputDimensionality=Customize  OutputDimensions=[3,4]
  Reshape2 : Reshape  OutputDimensionality=Customize  OutputDimensions=[3,4]
  Sum : Sum  Inputs=|+-
  VehSusp : Outport  VectorParamsAs1DForOutWhenUnconnected=off
  wires:
  Reshape1/1 -> Sum/1
  Mux2/1 -> Reshape1/1
  Veh/1 -> Bus Selector1/1, Bus Selector2/1
  Sum/1 -> Bus Creator3/1  "P"
  Inertial Frame CG to Axle Offset/1 -> Sum/2
  Mux1/1 -> Reshape2/1
  Bus Selector2/12 -> Mux1/12  "<zdot>"
  Bus Selector2/11 -> Mux1/11  "<ydot>"
  Bus Selector2/10 -> Mux1/10  "<xdot>"
  Bus Selector2/9 -> Mux1/9  "<zdot>"
  Bus Selector2/8 -> Mux1/8  "<ydot>"
  Bus Selector2/7 -> Mux1/7  "<xdot>"
  Bus Selector2/6 -> Mux1/6  "<zdot>"
  Bus Selector2/5 -> Mux1/5  "<ydot>"
  Bus Selector2/4 -> Mux1/4  "<xdot>"
  Bus Selector2/3 -> Mux1/3  "<zdot>"
  Bus Selector2/2 -> Mux1/2  "<ydot>"
  Bus Selector2/1 -> Mux1/1  "<xdot>"
  Bus Selector1/12 -> Mux2/12  "<Z>"
  Bus Selector1/11 -> Mux2/11  "<Y>"
  Bus Selector1/10 -> Mux2/10  "<X>"
  Bus Selector1/9 -> Mux2/9  "<Z>"
  Bus Selector1/8 -> Mux2/8  "<Y>"
  Bus Selector1/7 -> Mux2/7  "<X>"
  Bus Selector1/6 -> Mux2/6  "<Z>"
  Bus Selector1/5 -> Mux2/5  "<Y>"
  Bus Selector1/4 -> Mux2/4  "<X>"
  Bus Selector1/3 -> Mux2/3  "<Z>"
  Bus Selector1/2 -> Mux2/2  "<Y>"
  Bus Selector1/1 -> Mux2/1  "<X>"
  Bus Creator3/1 -> VehSusp/1  "Veh"
  Reshape2/1 -> Bus Creator3/2  "V"

== system EV6_LUT_FourWheel_EV6Battery77p4kWh_PowerCorrected/Vehicle Under Test1/Vehicle/Vehicle Dynamics/Vehicle 14DOF/Suspension/Double Wishbone Suspension/Wheel  Adapter ==
  Wheels : Inport
  Bus Selector : BusSelector  OutputSignals=TireFrame.Fx,TireFrame.Fy
  Bus Selector1 : BusSelector  OutputSignals=TireFrame.Re
  Bus Selector2 : BusSelector  OutputSignals=TireFrame.Mx,TireFrame.My,TireFrame.Mz
  Bus Selector3 : BusSelector  OutputSignals=TireFrame.z,TireFrame.zdot
  Matrix Concatenate : Concatenate  NumInputs=3  Mode=Multidimensional array
  Reshape{,1..7} (8 alike) : Reshape  OutputDimensionality=Row vector (2-D)
  WhlFx : Outport  VectorParamsAs1DForOutWhenUnconnected=off
  WhlFy : Outport  Port=2  VectorParamsAs1DForOutWhenUnconnected=off
  z : Outport  Port=3  VectorParamsAs1DForOutWhenUnconnected=off
  zdot : Outport  Port=4  VectorParamsAs1DForOutWhenUnconnected=off
  M : Outport  Port=5  VectorParamsAs1DForOutWhenUnconnected=off
  Re : Outport  Port=6  VectorParamsAs1DForOutWhenUnconnected=off
  wires:
  Reshape/1 -> z/1  "z"
  Matrix Concatenate/1 -> M/1  "M"
  Reshape5/1 -> Matrix Concatenate/3
  Reshape4/1 -> Matrix Concatenate/2
  Reshape3/1 -> Matrix Concatenate/1
  Bus Selector2/3 -> Reshape5/1  "<Mz>"
  Bus Selector2/2 -> Reshape4/1  "<My>"
  Bus Selector2/1 -> Reshape3/1  "<Mx>"
  Reshape1/1 -> Re/1  "Re"
  Bus Selector1/1 -> Reshape1/1  "<Re>"
  Reshape2/1 -> zdot/1  "zdot"
  Bus Selector3/2 -> Reshape2/1  "<zdot>"
  Wheels/1 -> Bus Selector/1, Bus Selector3/1, Bus Selector2/1, Bus Selector1/1
  Bus Selector3/1 -> Reshape/1  "<z>"
  Bus Selector/2 -> Reshape7/1  "<Fy>"
  Bus Selector/1 -> Reshape6/1  "<Fx>"
  Reshape6/1 -> WhlFx/1
  Reshape7/1 -> WhlFy/1

== system EV6_LUT_FourWheel_EV6Battery77p4kWh_PowerCorrected/Vehicle Under Test1/Vehicle/Vehicle Dynamics/Vehicle 14DOF/Suspension/Independent Mapped Front Suspension Mapped Solid Axle Rear Suspension/Steer Rate Adapter ==
  Veh : Inport
  Add : Sum
  Bus Selector3 : BusSelector  OutputSignals=BdyFrm.Cg.AngVel.r
  Constant : Constant  Value=zeros(1,4)
  Matrix Concatenate : Concatenate  NumInputs=3  Mode=Multidimensional array
  Matrix Concatenate1 : Concatenate  NumInputs=3  Mode=Multidimensional array
  Reshape2 : Reshape  OutputDimensionality=Row vector (2-D)
  Reshape3 : Reshape  OutputDimensionality=Row vector (2-D)
  Reshape4 : Reshape  OutputDimensionality=Row vector (2-D)
  Selector3 : Selector  InputPortWidth=1  IndexOptions=Index vector (dialog)  Indices=[1 1 1 1]  OutputSizes=1
  SteerRates : Constant  Value=zeros(1,4)
  AngVel : Outport  VectorParamsAs1DForOutWhenUnconnected=off
  wires:
  Add/1 -> AngVel/1  "AngVel"
  Veh/1 -> Bus Selector3/1
  Matrix Concatenate1/1 -> Add/1
  Reshape3/1 -> Matrix Concatenate/1, Matrix Concatenate/2
  Reshape4/1 -> Matrix Concatenate/3
  SteerRates/1 -> Reshape2/1
  Matrix Concatenate/1 -> Add/2
  Bus Selector3/1 -> Selector3/1  "<r>"
  Selector3/1 -> Reshape4/1
  Constant/1 -> Reshape3/1
  Reshape2/1 -> Matrix Concatenate1/2, Matrix Concatenate1/3, Matrix Concatenate1/1

== system EV6_LUT_FourWheel_EV6Battery77p4kWh_PowerCorrected/Vehicle Under Test1/Vehicle/Vehicle Dynamics/Vehicle 14DOF/Suspension/Independent Mapped Front Suspension Mapped Solid Axle Rear Suspension/Steering Adapter ==
  Steer : Inport
  Reshape1 : Reshape  OutputDimensionality=Row vector (2-D)
  Selector : Selector  IndexOptions=Index vector (dialog)  Indices=[1 2]  OutputSizes=1
  StrgAng : Outport  VectorParamsAs1DForOutWhenUnconnected=off
  wires:
  Selector/1 -> Reshape1/1
  Steer/1 -> Selector/1
  Reshape1/1 -> StrgAng/1

== system EV6_LUT_FourWheel_EV6Battery77p4kWh_PowerCorrected/Vehicle Under Test1/Vehicle/Vehicle Dynamics/Vehicle 14DOF/Suspension/Independent Mapped Front Suspension Mapped Solid Axle Rear Suspension/Vehicle Adapter ==
  Veh : Inport
  Bus Creator3 : BusCreator  Inputs=2
  Bus Selector1 : BusSelector  OutputSignals=InertFrm.FrntAxl.Lft.Disp.X,InertFrm.FrntAxl.Lft.Disp.Y,InertFrm.FrntAxl.Lft.Disp.Z,InertFrm.FrntAxl.Rght.Disp.X,InertFrm.FrntAxl.Rght.Disp.Y,InertFrm.FrntAxl.Rght.Disp.Z,InertFrm.RearAxl.Lft.Disp.X,InertFrm.RearAxl.Lft.Disp.Y,InertFrm.RearAxl.Lft.Disp.Z,InertFrm.RearAxl.Rght.Disp.X,InertFrm.RearAxl.Rght.Disp.Y,InertFrm.RearAxl.Rght.Disp.Z
  Bus Selector2 : BusSelector  OutputSignals=BdyFrm.FrntAxl.Lft.Vel.xdot,BdyFrm.FrntAxl.Lft.Vel.ydot,BdyFrm.FrntAxl.Lft.Vel.zdot,BdyFrm.FrntAxl.Rght.Vel.xdot,BdyFrm.FrntAxl.Rght.Vel.ydot,BdyFrm.FrntAxl.Rght.Vel.zdot,BdyFrm.RearAxl.Lft.Vel.xdot,BdyFrm.RearAxl.Lft.Vel.ydot,BdyFrm.RearAxl.Lft.Vel.zdot,BdyFrm.RearAxl.Rght.Vel.xdot,BdyFrm.RearAxl.Rght.Vel.ydot,BdyFrm.RearAxl.Rght.Vel.zdot
  Inertial Frame CG to Axle Offset : Constant  Value=[zeros(2,4);h*ones(1,4)]
  Mux1 : Mux  Inputs=12
  Mux2 : Mux  Inputs=12
  Reshape : Reshape  OutputDimensionality=Customize  OutputDimensions=[3,4]
  Reshape2 : Reshape  OutputDimensionality=Customize  OutputDimensions=[3,4]
  Sum : Sum  Inputs=|+-
  VehSusp : Outport  VectorParamsAs1DForOutWhenUnconnected=off
  wires:
  Sum/1 -> Bus Creator3/1  "P"
  Inertial Frame CG to Axle Offset/1 -> Sum/2
  Mux2/1 -> Reshape/1
  Mux1/1 -> Reshape2/1
  Bus Selector2/12 -> Mux1/12  "<zdot>"
  Bus Selector2/11 -> Mux1/11  "<ydot>"
  Bus Selector2/10 -> Mux1/10  "<xdot>"
  Bus Selector2/9 -> Mux1/9  "<zdot>"
  Bus Selector2/8 -> Mux1/8  "<ydot>"
  Bus Selector2/7 -> Mux1/7  "<xdot>"
  Bus Selector2/6 -> Mux1/6  "<zdot>"
  Bus Selector2/5 -> Mux1/5  "<ydot>"
  Bus Selector2/4 -> Mux1/4  "<xdot>"
  Bus Selector2/3 -> Mux1/3  "<zdot>"
  Bus Selector2/2 -> Mux1/2  "<ydot>"
  Bus Selector2/1 -> Mux1/1  "<xdot>"
  Bus Selector1/12 -> Mux2/12  "<Z>"
  Bus Selector1/11 -> Mux2/11  "<Y>"
  Bus Selector1/10 -> Mux2/10  "<X>"
  Bus Selector1/9 -> Mux2/9  "<Z>"
  Bus Selector1/8 -> Mux2/8  "<Y>"
  Bus Selector1/7 -> Mux2/7  "<X>"
  Bus Selector1/6 -> Mux2/6  "<Z>"
  Bus Selector1/5 -> Mux2/5  "<Y>"
  Bus Selector1/4 -> Mux2/4  "<X>"
  Bus Selector1/3 -> Mux2/3  "<Z>"
  Bus Selector1/2 -> Mux2/2  "<Y>"
  Bus Selector1/1 -> Mux2/1  "<X>"
  Reshape/1 -> Sum/1
  Bus Creator3/1 -> VehSusp/1  "Veh"
  Reshape2/1 -> Bus Creator3/2  "V"
  Veh/1 -> Bus Selector1/1, Bus Selector2/1

== system EV6_LUT_FourWheel_EV6Battery77p4kWh_PowerCorrected/Vehicle Under Test1/Vehicle/Vehicle Dynamics/Vehicle 14DOF/Suspension/Independent Mapped Front Suspension Mapped Solid Axle Rear Suspension/Wheel  Adapter ==
  Wheels : Inport
  Bus Selector : BusSelector  OutputSignals=TireFrame.Fx,TireFrame.Fy
  Bus Selector1 : BusSelector  OutputSignals=TireFrame.Re
  Bus Selector2 : BusSelector  OutputSignals=TireFrame.Mx,TireFrame.My,TireFrame.Mz
  Bus Selector3 : BusSelector  OutputSignals=TireFrame.z,TireFrame.zdot
  Matrix Concatenate : Concatenate  NumInputs=3  Mode=Multidimensional array
  Reshape{,1..7} (8 alike) : Reshape  OutputDimensionality=Row vector (2-D)
  WhlFx : Outport  VectorParamsAs1DForOutWhenUnconnected=off
  WhlFy : Outport  Port=2  VectorParamsAs1DForOutWhenUnconnected=off
  z : Outport  Port=3  VectorParamsAs1DForOutWhenUnconnected=off
  zdot : Outport  Port=4  VectorParamsAs1DForOutWhenUnconnected=off
  M : Outport  Port=5  VectorParamsAs1DForOutWhenUnconnected=off
  Re : Outport  Port=6  VectorParamsAs1DForOutWhenUnconnected=off
  wires:
  Reshape/1 -> z/1  "z"
  Matrix Concatenate/1 -> M/1  "M"
  Reshape5/1 -> Matrix Concatenate/3
  Reshape4/1 -> Matrix Concatenate/2
  Reshape3/1 -> Matrix Concatenate/1
  Bus Selector2/3 -> Reshape5/1  "<Mz>"
  Bus Selector2/2 -> Reshape4/1  "<My>"
  Bus Selector2/1 -> Reshape3/1  "<Mx>"
  Reshape1/1 -> Re/1  "Re"
  Bus Selector1/1 -> Reshape1/1  "<Re>"
  Reshape2/1 -> zdot/1  "zdot"
  Bus Selector3/2 -> Reshape2/1  "<zdot>"
  Wheels/1 -> Bus Selector/1, Bus Selector3/1, Bus Selector2/1, Bus Selector1/1
  Bus Selector3/1 -> Reshape/1  "<z>"
  Bus Selector/2 -> Reshape7/1  "<Fy>"
  Bus Selector/1 -> Reshape6/1  "<Fx>"
  Reshape6/1 -> WhlFx/1
  Reshape7/1 -> WhlFy/1

== system EV6_LUT_FourWheel_EV6Battery77p4kWh_PowerCorrected/Vehicle Under Test1/Vehicle/Vehicle Dynamics/Vehicle 14DOF/Suspension/MacPherson Front Suspension Solid Axle Rear Suspension/Steer Rate Adapter ==
  Veh : Inport
  Add : Sum
  Bus Selector3 : BusSelector  OutputSignals=BdyFrm.Cg.AngVel.r
  Constant : Constant  Value=zeros(1,4)
  Matrix Concatenate : Concatenate  NumInputs=3  Mode=Multidimensional array
  Matrix Concatenate1 : Concatenate  NumInputs=3  Mode=Multidimensional array
  Reshape2 : Reshape  OutputDimensionality=Row vector (2-D)
  Reshape3 : Reshape  OutputDimensionality=Row vector (2-D)
  Reshape4 : Reshape  OutputDimensionality=Row vector (2-D)
  Selector3 : Selector  InputPortWidth=1  IndexOptions=Index vector (dialog)  Indices=[1 1 1 1]  OutputSizes=1
  SteerRates : Constant  Value=zeros(1,4)
  AngVel : Outport  VectorParamsAs1DForOutWhenUnconnected=off
  wires:
  Add/1 -> AngVel/1  "AngVel"
  Veh/1 -> Bus Selector3/1
  Matrix Concatenate1/1 -> Add/1
  Reshape3/1 -> Matrix Concatenate/1, Matrix Concatenate/2
  Reshape4/1 -> Matrix Concatenate/3
  SteerRates/1 -> Reshape2/1
  Matrix Concatenate/1 -> Add/2
  Bus Selector3/1 -> Selector3/1  "<r>"
  Selector3/1 -> Reshape4/1
  Constant/1 -> Reshape3/1
  Reshape2/1 -> Matrix Concatenate1/2, Matrix Concatenate1/3, Matrix Concatenate1/1

== system EV6_LUT_FourWheel_EV6Battery77p4kWh_PowerCorrected/Vehicle Under Test1/Vehicle/Vehicle Dynamics/Vehicle 14DOF/Suspension/MacPherson Front Suspension Solid Axle Rear Suspension/Steering Adapter ==
  Steer : Inport
  Reshape1 : Reshape  OutputDimensionality=Row vector (2-D)
  Selector : Selector  IndexOptions=Index vector (dialog)  Indices=[1 2]  OutputSizes=1
  StrgAng : Outport  VectorParamsAs1DForOutWhenUnconnected=off
  wires:
  Selector/1 -> Reshape1/1
  Steer/1 -> Selector/1
  Reshape1/1 -> StrgAng/1
